simulink model "grid_afe_n"  (R2026a)
settings: Solver=ode23tb  StopTime=simlength  FixedStep=tc  MaxStep=glb_time.tc
values from neighbouring files (symbols this model uses):
  afe_ctrl = ctrl_afe_setup(glb_time.ts_afe, grid_emu.omega_grid_nom)    [init_model.m]
  afe_pwm_phase_shift_mod1 = 0    [init_model.m]
  afe_pwm_phase_shift_mod2 = 0    [init_model.m]
  afe_pwm_phase_shift_mod3 = 0    [init_model.m]
  afe_pwm_phase_shift_mod4 = 0    [init_model.m]
  filters = setup_global_filters(glb_time.ts_afe, glb_time.ts_inv, glb_time.ts_dab, glb_time.tc)    [init_model.m]
  frt_data = frt_settings(test_index, test_subindex, asymmetric_error_type,      enable_frt_1, enable_frt_2, start_time_LVRT, deepPOSxi, deepPOSeta, deepNEGxi, deepNEGeta)    [init_model.m]
  glb_time = timing_setup(fpwm_afe, trgo_afe, fpwm_inv, trgo_inv, fpwm_single_phase_inv, trgo_single_phase_inv, fpwm_dab, trgo_dab,      fpwm_psfbc, trgo_psfbc, fpwm_isop_rail, trgo_isop_rail, fpwm_cllc, trgo_cllc, t_measure, tc_factor, tc_decimation, delay_pwm, dead_time_afe,      dead_time_inv, dead_time_single_phase_inv, dead_time_dab, dead_time_psfbc, dead_time_isop_rail, dead_time_cllc)    [init_model.m]
  grid_emu = grid_three_phase_emulator('Dyn11', delta_star, grid_nominal_power, application_voltage, us1, us2, fgrid,                  eq_grid_inductance, eq_grid_resistance, eta, ucc, i1m, p_iron, n1, n2, core_area, core_length, mur,                  up_xi_pu_ref, up_eta_pu_ref, un_xi_pu_ref, un_eta_pu_ref)    [init_model.m]
  i_react_pos_ref_2 = -ixi_ref_mod1*tan(acos(0.95))    [init_model.m]
  i_react_pos_ref_3 = ixi_ref_mod1*tan(acos(0.95))    [init_model.m]
  ixi_ref_mod1 = -0.85    [init_model.m]
  ixi_ref_mod2 = -0.85    [init_model.m]
  ixi_ref_mod3 = -0.85    [init_model.m]
  ixi_ref_mod4 = -0.85    [init_model.m]
  ki_align = 18    [init_model.m]
  kp_align = 0.25    [init_model.m]
  lim_down_align = -0.05    [init_model.m]
  lim_up_align = 0.05    [init_model.m]
  mavarage_filter_frequency_base_order = 2    [init_model.m]
  time_gain_afe_module_1 = 1.0002    [init_model.m]
  time_gain_afe_module_2 = 1.0015    [init_model.m]
  time_gain_afe_module_3 = 0.9988    [init_model.m]
  time_gain_afe_module_4 = 1.0020    (= 1.002)    [init_model.m]
  time_i_react_pos_ref_1 = start_time_LVRT + error_length + 0.335    [init_model.m]
  time_i_react_pos_ref_2 = time_i_react_pos_ref_1 + 0.5    (= 0.5)    [init_model.m]
  u_cm_comp_mod1 = 0    [init_model.m]
  u_cm_comp_mod2 = -1    [init_model.m]
  u_cm_comp_mod3 = -1    [init_model.m]
  u_cm_comp_mod4 = -1    [init_model.m]
undefined symbols (not defined in the file or in its folder): hwdata, magnitude
libraries: fl_lib x113, nesl_utility x75, moving_average_filter x40, moving_average_filter_cc x32, sl_discontinuities x12, linear_double_integrator_observer_ccaller x8, discrete_time_low_pass_filter x4, threephase_inductor_lib x4, dclink_for_two_levels x4, three_phase_pwm_modulator x4, three_phase_inverter_ideal_switch_based_model x4, three_phase_inverter_igbt_advanced_thermal_model x4
(part 18 of 19)

== matlab function grid_afe_n/afe_abc_mod4/AFE_control/afe_control/FRT-VDE4110/FRT-Detection/LVRT_detector ==
  data: vxi_p input; vxi_n input; veta_n input; vxi_p_dot input; vxi_n_dot input; enable input; red_dyn_enabled input; pwr_lim_enable output; frt_exceeded output; reset input; frt_active output; frt_state output; red_dyn_active output
function [pwr_lim_enable, frt_exceeded, frt_active, frt_state, red_dyn_active]  = lvrt_detector(vxi_p,vxi_n,veta_n,vxi_p_dot,vxi_n_dot, enable, red_dyn_enabled, reset)

    persistent state count count2 state_pwr_lim
    
    LVRT_IDLE = 0;
    LVRT_ACTIVE = 1;
    LVRT_EXCEEDED = 2;
    
    PWR_LIM_DISABLED = 0;
    PWR_LIM_ENABLED  = 1;
    
    LVRT_VPOS_TH_LOW			= 0.85;
    LVRT_VPOS_TH_HIGH			= 1.15;
    LVRT_SEQ_DETECTION_HYST		= 0.1;
    LVRT_VNEG_TH				= 0.1;
    LVRT_VPOS_DOT_TH			= 2.0;
    LVRT_VNEG_DOT_TH			= 2.0;
    LVRT_VPOS_PWRLIM_TH			= 0.8;
    LVRT_VNEG_PWRLIM_TH			= 0.1;
    LVRT_PWRLIM_HYST			= 0.1;
    LVRT_VPOS_RED_DYN_TH        = 0.7;
    LVRT_VNEG_RED_DYN_TH        = 0.2;
    LVRT_TIME_HOLD_MAX          = 61000;
    
    RED_DYN_NOT_ACTIVE = 0;
    RED_DYN_ACTIVE     = 1;
        
    if isempty(state)
        state = LVRT_IDLE;
        state_pwr_lim = PWR_LIM_DISABLED;
        count = 0;
        count2 = 0;
    end

    vn = sqrt(vxi_n^2+veta_n^2);

    if enable == 1
        
        switch state
            
            case LVRT_IDLE
                if ((vxi_p > LVRT_VPOS_TH_HIGH || vxi_p < LVRT_VPOS_TH_LOW || vn > LVRT_VNEG_TH) ...
                     && (vxi_p_dot > LVRT_VPOS_DOT_TH || vxi_n_dot > LVRT_VNEG_DOT_TH) && ...
                     count2 > 1000)
                    state = LVRT_ACTIVE;
                end
                frt_active = 0;
                frt_exceeded = 0;
                count = 0;
                frt_state = LVRT_IDLE;
                state_pwr_lim = PWR_LIM_DISABLED;                  
                red_dyn_active = RED_DYN_NOT_ACTIVE;
                count2 = count2 + 1;

            case LVRT_ACTIVE
                count2 = 0;
                % LVRT condition not active anymore
                if (vxi_p >= LVRT_VPOS_TH_LOW  + LVRT_SEQ_DETECTION_HYST && ...
                    vxi_p <  LVRT_VPOS_TH_HIGH - LVRT_SEQ_DETECTION_HYST)
                    state = LVRT_IDLE;
                % LVRT exceeded
                elseif (count >= LVRT_TIME_HOLD_MAX)
                    state = LVRT_EXCEEDED;
                end
                
                % handle power limitation
                if (vxi_p < LVRT_VPOS_PWRLIM_TH || vn > LVRT_VNEG_PWRLIM_TH) 
                    state_pwr_lim = PWR_LIM_ENABLED;
                elseif (vxi_p > LVRT_VPOS_PWRLIM_TH + LVRT_PWRLIM_HYST && vn < LVRT_VPOS_PWRLIM_TH - LVRT_PWRLIM_HYST)
                    state_pwr_lim = PWR_LIM_DISABLED;                  
                end
                
                % handle reduced dynamic grid support
                if red_dyn_enabled && (vxi_p < LVRT_VPOS_RED_DYN_TH || vn > LVRT_VNEG_RED_DYN_TH)
                    red_dyn_active = RED_DYN_ACTIVE;
                else
                    red_dyn_active = RED_DYN_NOT_ACTIVE;
                end
                 
                frt_active = 1;
                frt_exceeded = 0;
                frt_state = LVRT_ACTIVE;
                
                count = count + 1;
            
            case LVRT_EXCEEDED

                if ((reset == 1) || (enable == 0))
                    state = LVRT_IDLE;
                else
                    state = LVRT_EXCEEDED;
                end
                
                frt_exceeded = 1;
                frt_active = 0; 
                frt_state = LVRT_EXCEEDED;
                red_dyn_active = RED_DYN_NOT_ACTIVE;
            
            otherwise
                state = LVRT_IDLE;
                frt_active = 0;
                frt_exceeded = 0;
                frt_state = LVRT_IDLE;
                red_dyn_active = RED_DYN_NOT_ACTIVE;
        end
        
        if state_pwr_lim == PWR_LIM_ENABLED
            pwr_lim_enable = 1;
        else
            pwr_lim_enable = 0;
        end      
    else
        state = LVRT_IDLE;
        frt_active = 0;
        pwr_lim_enable = 0;
        frt_exceeded = 0;
        frt_state = LVRT_IDLE;
        red_dyn_active = RED_DYN_NOT_ACTIVE;
    end
end

== matlab function grid_afe_n/afe_abc_mod1/AFE_control/afe_control/current_ctrl/current_transformation/alphabeta2xieta ==
  data: alpha input; xi output; beta input; gamma input; eta output
function [xi,eta] = alphabeta2xieta(alpha,beta,gamma)

    xi  =  alpha*cos(gamma) + beta*sin(gamma);
    eta = -alpha*sin(gamma) + beta*cos(gamma);

end

== matlab function grid_afe_n/afe_abc_mod4/AFE_control/afe_control/FRT-VDE4110/FRT-PosNegReactiveCurrentReferences/avg_flt_500ms/avg_flt_1 ==
  data: x input; y1 output; w input; ts input; enable input
function y1  = avg_flt(x,w,ts, enable)

    persistent x_int x_int_1 y_N N

    N = (1/(w/(2*pi)))/ts+1;

    if isempty(x_int)
        x_int_1 = 0;
        y_N = zeros(1,N);
        y1 = 0;
    end


    if enable == 1
        x_int = x * ts * w + x_int_1;
        x_int_1 = x_int;
        y_N(1,1) = x_int;
        y1 = 1/(2*pi)*((y_N(1,1) - y_N(1,N)));
        for i = 1:(N-1)
            y_N(1,N+1-i) = y_N(1,N-i); 
        end
    else
        y1 = 1/(2*pi)*((y_N(1,1) - y_N(1,N)));
    end
end

== matlab function grid_afe_n/afe_abc_mod4/AFE_control/afe_control/FRT-VDE4110/FRT-PosNegReactiveCurrentReferences/avg_flt_500ms1/avg_flt_1 ==
  data: x input; y1 output; w input; ts input; enable input
function y1  = avg_flt(x,w,ts, enable)

    persistent x_int x_int_1 y_N N

    N = (1/(w/(2*pi)))/ts+1;

    if isempty(x_int)
        x_int_1 = 0;
        y_N = zeros(1,N);
        y1 = 0;
    end


    if enable == 1
        x_int = x * ts * w + x_int_1;
        x_int_1 = x_int;
        y_N(1,1) = x_int;
        y1 = 1/(2*pi)*((y_N(1,1) - y_N(1,N)));
        for i = 1:(N-1)
            y_N(1,N+1-i) = y_N(1,N-i); 
        end
    else
        y1 = 1/(2*pi)*((y_N(1,1) - y_N(1,N)));
    end
end

== matlab function grid_afe_n/afe_abc_mod4/AFE_control/afe_control/FRT-VDE4110/FRT-PosNegReactiveCurrentReferences/avg_flt_500ms2/avg_flt_1 ==
  data: x input; y1 output; w input; ts input; enable input
function y1  = avg_flt(x,w,ts, enable)

    persistent x_int x_int_1 y_N N

    N = (1/(w/(2*pi)))/ts+1;

    if isempty(x_int)
        x_int_1 = 0;
        y_N = zeros(1,N);
        y1 = 0;
    end


    if enable == 1
        x_int = x * ts * w + x_int_1;
        x_int_1 = x_int;
        y_N(1,1) = x_int;
        y1 = 1/(2*pi)*((y_N(1,1) - y_N(1,N)));
        for i = 1:(N-1)
            y_N(1,N+1-i) = y_N(1,N-i); 
        end
    else
        y1 = 1/(2*pi)*((y_N(1,1) - y_N(1,N)));
    end
end

== matlab function grid_afe_n/afe_abc_mod4/AFE_control/afe_control/FRT-VDE4110/FRT-PosNegReactiveCurrentReferences/avg_flt_500ms3/avg_flt_1 ==
  data: x input; y1 output; w input; ts input; enable input
function y1  = avg_flt(x,w,ts, enable)

    persistent x_int x_int_1 y_N N

    N = (1/(w/(2*pi)))/ts+1;

    if isempty(x_int)
        x_int_1 = 0;
        y_N = zeros(1,N);
        y1 = 0;
    end


    if enable == 1
        x_int = x * ts * w + x_int_1;
        x_int_1 = x_int;
        y_N(1,1) = x_int;
        y1 = 1/(2*pi)*((y_N(1,1) - y_N(1,N)));
        for i = 1:(N-1)
            y_N(1,N+1-i) = y_N(1,N-i); 
        end
    else
        y1 = 1/(2*pi)*((y_N(1,1) - y_N(1,N)));
    end
end

== matlab function grid_afe_n/afe_abc_mod4/AFE_control/afe_control/current_ctrl/current_transformation/alphabeta2xieta ==
  data: alpha input; xi output; beta input; gamma input; eta output
function [xi,eta] = alphabeta2xieta(alpha,beta,gamma)

    xi  =  alpha*cos(gamma) + beta*sin(gamma);
    eta = -alpha*sin(gamma) + beta*cos(gamma);

end

== matlab function grid_afe_n/afe_abc_mod4/AFE_control/afe_control/current_ctrl/current_transformation/uvw2alphabeta ==
  data: u input; alpha output; v input; w input; beta output
function [alpha,beta] = uvw2alphabeta(u,v,w)

alpha = 2/3*(u - 1/2*v - 1/2*w);
beta  = 2/3*(sqrt(3)/2*(v - w));

end

== matlab function grid_afe_n/afe_abc_mod4/AFE_control/afe_control/current_ctrl/inner_current_ctrl/zero_current_ctrl/antiwind_up/MATLAB Function1 ==
  data: da input; das output; db input; dc input; scaling input; dbs output; dcs output
function [das, dbs, dcs] = fcn(da,db,dc,scaling)

das = da/scaling;
dbs = db/scaling;
dcs = dc/scaling;

== matlab function grid_afe_n/afe_abc_mod4/AFE_control/afe_control/current_ctrl/inner_current_ctrl/zero_current_ctrl/antiwind_up/MATLAB Function2 ==
  data: a input; alpha output; b input; c input; beta output; gamma output
function [alpha,beta, gamma] = abc2alphabeta(a,b,c)

alpha = 2/3*(a - 1/2*b - 1/2*c);
beta  = 1/sqrt(3)*(b - c);
gamma = (a+b+c)/3;

end

== matlab function grid_afe_n/afe_abc_mod4/AFE_control/afe_control/current_ctrl/xieta2abc/MATLAB Function2 ==
  data: alpha input; a output; beta input; b output; c output
function [a,b,c] = alphabeta2abc(alpha,beta)

a = alpha;
b = -(1/2)*alpha + sqrt(3)/2*beta;
c = -(1/2)*alpha - sqrt(3)/2*beta;

end

== matlab function grid_afe_n/afe_abc_mod4/AFE_control/afe_control/current_ctrl/xieta2abc/Negative Sequence ==
  data: xi input; alpha output; eta input; phase input; beta output
function [alpha,beta] = neg2alphabeta(xi,eta,phase)

    alpha = xi*cos(phase)  + eta*sin(phase);
    beta  = -xi*sin(phase) + eta*cos(phase);

end

== matlab function grid_afe_n/afe_abc_mod1/AFE_control/afe_control/grid_voltage_phase_lock_loops/FHT-PLL/pll_stageB/double_integrator_observer/bounder1 ==
  data: u input; y output
function y = bounder(u)
    
    y = -pi + mod(u+3*pi,2*pi);
    
end

== matlab function grid_afe_n/afe_abc_mod4/AFE_control/afe_control/current_ctrl/xieta2abc/Positive Sequence ==
  data: xi input; alpha output; eta input; phase input; beta output
function [alpha,beta] = pos2alphabeta(xi,eta,phase)

    alpha = xi*cos(phase) - eta*sin(phase);
    beta  = xi*sin(phase) + eta*cos(phase);

end

== matlab function grid_afe_n/afe_abc_mod4/AFE_control/afe_control/grid_current_sequences_and_reactive_pwr_ctrl/grid_current_sampling_and_alpha_beta_transformation/i_abc2alphabeta ==
  data: i_abc input; alpha output; beta output
function [alpha,beta] = abc2alphabeta(i_abc)

alpha = 2/3*(i_abc(1) - 1/2*i_abc(2) - 1/2*i_abc(3));
beta  = 1/sqrt(3)*(i_abc(2) - i_abc(3));

end

== matlab function grid_afe_n/afe_abc_mod4/AFE_control/afe_control/grid_current_sequences_and_reactive_pwr_ctrl/i_alphabeta2xieta/MATLAB Function ==
  data: alpha input; xi output; beta input; gamma input; eta output
function [xi,eta] = alphabeta2pos(alpha,beta,gamma)

    xi  =  alpha*cos(gamma) + beta*sin(gamma);
    eta = -alpha*sin(gamma) + beta*cos(gamma);

end

== matlab function grid_afe_n/afe_abc_mod4/AFE_control/afe_control/grid_current_sequences_and_reactive_pwr_ctrl/i_alphabeta2xieta/MATLAB Function1 ==
  data: alpha input; xi output; beta input; gamma input; eta output
function [xi,eta] = alphabeta2neg(alpha,beta,gamma)

    xi  = alpha*cos(gamma) - beta*sin(gamma);
    eta = alpha*sin(gamma) + beta*cos(gamma);

end

== matlab function grid_afe_n/afe_abc_mod4/AFE_control/afe_control/grid_voltage_phase_lock_loops/FHT-PLL/pll_stageA/filter_and_transformation/abc2alphabeta ==
  data: a input; alpha output; b input; c input; beta output
function [alpha,beta] = abc2alphabeta(a,b,c)

alpha = 2/3*(a - 1/2*b - 1/2*c);
beta  = 1/sqrt(3)*(b - c);

end

== matlab function grid_afe_n/afe_abc_mod4/AFE_control/afe_control/grid_voltage_phase_lock_loops/FHT-PLL/pll_stageA/sequences/alphabeta2xieta ==
  data: alpha input; xi output; beta input; gamma input; eta output
function [xi,eta] = alphabeta2xieta_pos(alpha,beta,gamma)

    xi  =  (alpha*cos(gamma) + beta*sin(gamma));
    eta = (-alpha*sin(gamma) + beta*cos(gamma));

end

== matlab function grid_afe_n/afe_abc_mod4/AFE_control/afe_control/grid_voltage_phase_lock_loops/FHT-PLL/pll_stageB/bounder1 ==
  data: u input; y output
function y = bounder(u)
    y = -pi + mod(u+3*pi,2*pi);
end

== matlab function grid_afe_n/afe_abc_mod2/AFE_control/afe_control/FRT-VDE4110/FRT-PosNegReactiveCurrentReferences/avg_flt_500ms/avg_flt_1 ==
  data: x input; y1 output; w input; ts input; enable input
function y1  = avg_flt(x,w,ts, enable)

    persistent x_int x_int_1 y_N N

    N = (1/(w/(2*pi)))/ts+1;

    if isempty(x_int)
        x_int_1 = 0;
        y_N = zeros(1,N);
        y1 = 0;
    end


    if enable == 1
        x_int = x * ts * w + x_int_1;
        x_int_1 = x_int;
        y_N(1,1) = x_int;
        y1 = 1/(2*pi)*((y_N(1,1) - y_N(1,N)));
        for i = 1:(N-1)
            y_N(1,N+1-i) = y_N(1,N-i); 
        end
    else
        y1 = 1/(2*pi)*((y_N(1,1) - y_N(1,N)));
    end
end

== matlab function grid_afe_n/afe_abc_mod4/AFE_control/afe_control/grid_voltage_phase_lock_loops/FHT-PLL/pll_stageB/double_integrator_observer/bounder1 ==
  data: u input; y output
function y = bounder(u)
    
    y = -pi + mod(u+3*pi,2*pi);
    
end

== matlab function grid_afe_n/afe_abc_mod4/AFE_control/afe_control/grid_voltage_phase_lock_loops/FHT-PLL/pll_stageB/double_integrator_observer/bounder2 ==
  data: u input; y output
function y = bounder(u)
    
    y = -pi + mod(u+3*pi,2*pi);
    
end

== matlab function grid_afe_n/afe_abc_mod4/AFE_control/afe_control/grid_voltage_phase_lock_loops/dq_pll/pll_stageA/mormalization_and_transformation/abc2alphabeta ==
  data: a input; alpha output; b input; c input; beta output
function [alpha,beta] = abc2alphabeta(a,b,c)

alpha = 2/3*(a - 1/2*b - 1/2*c);
beta  = 1/sqrt(3)*(b - c);

end

== matlab function grid_afe_n/afe_abc_mod4/AFE_control/afe_control/grid_voltage_phase_lock_loops/dq_pll/pll_stageA/sequences/alphabeta2xieta/alphabeta2xieta_neg ==
  data: alpha input; xi output; beta input; gamma input; eta output
function [xi,eta] = alphabeta2xieta_neg(alpha,beta,gamma)

    xi  = alpha*cos(gamma) - beta*sin(gamma);
    eta = alpha*sin(gamma) + beta*cos(gamma);

end

== matlab function grid_afe_n/afe_abc_mod4/AFE_control/afe_control/grid_voltage_phase_lock_loops/dq_pll/pll_stageA/sequences/alphabeta2xieta/alphabeta2xieta_pos ==
  data: alpha input; xi output; beta input; gamma input; eta output
function [xi,eta] = alphabeta2xieta_pos(alpha,beta,gamma)

    xi  =  alpha*cos(gamma) + beta*sin(gamma);
    eta = -alpha*sin(gamma) + beta*cos(gamma);

end

== matlab function grid_afe_n/afe_abc_mod4/AFE_control/afe_control/grid_voltage_phase_lock_loops/dq_pll/pll_stageB/bounder1 ==
  data: u input; y output
function y = bounder(u)
    y = -pi + mod(u+3*pi,2*pi);
end

== matlab function grid_afe_n/afe_abc_mod4/AFE_control/afe_control/grid_voltage_phase_lock_loops/dq_pll/pll_stageB/double_integrator_observer/bounder1 ==
  data: u input; y output
function y = bounder(u)
    
    y = -pi + mod(u+3*pi,2*pi);
    
end

== matlab function grid_afe_n/afe_abc_mod4/AFE_control/afe_control/grid_voltage_phase_lock_loops/dq_pll/pll_stageB/double_integrator_observer/bounder2 ==
  data: u input; y output
function y = bounder(u)
    
    y = -pi + mod(u+3*pi,2*pi);
    
end

== matlab function grid_afe_n/afe_abc_mod4/AFE_control/afe_control/grid_voltage_sequences/grid_voltage_sampling_and_alpha_beta_transformation/v_abc2alphabeta ==
  data: v_abc input; alpha output; beta output
function [alpha,beta] = abc2alphabeta(v_abc)

alpha = 2/3*(v_abc(1) - 1/2*v_abc(2) - 1/2*v_abc(3));
beta  = 1/sqrt(3)*(v_abc(2) - v_abc(3));

end

== matlab function grid_afe_n/afe_abc_mod4/AFE_control/afe_control/grid_voltage_sequences/v_alphabeta2xieta/MATLAB Function ==
  data: alpha input; xi output; beta input; gamma input; eta output
function [xi,eta] = alphabeta2pos(alpha,beta,gamma)

    xi  =  alpha*cos(gamma) + beta*sin(gamma);
    eta = -alpha*sin(gamma) + beta*cos(gamma);

end

== matlab function grid_afe_n/afe_abc_mod4/AFE_control/afe_control/grid_voltage_sequences/v_alphabeta2xieta/MATLAB Function1 ==
  data: alpha input; xi output; beta input; gamma input; eta output
function [xi,eta] = alphabeta2neg(alpha,beta,gamma)

    xi  = alpha*cos(gamma) - beta*sin(gamma);
    eta = alpha*sin(gamma) + beta*cos(gamma);

end

== matlab function grid_afe_n/afe_abc_mod4/AFE_control/afe_control/islanding_mode_detector/MATLAB Function ==
  data: alpha input; xi output; beta input; gamma input; eta output
function [xi,eta] = alphabeta2pos(alpha,beta,gamma)

    xi  =  alpha*cos(gamma) + beta*sin(gamma);
    eta = -alpha*sin(gamma) + beta*cos(gamma);

end

== matlab function grid_afe_n/afe_abc_mod2/AFE_control/afe_control/FRT-VDE4110/FRT-PosNegReactiveCurrentReferences/avg_flt_500ms1/avg_flt_1 ==
  data: x input; y1 output; w input; ts input; enable input
function y1  = avg_flt(x,w,ts, enable)

    persistent x_int x_int_1 y_N N

    N = (1/(w/(2*pi)))/ts+1;

    if isempty(x_int)
        x_int_1 = 0;
        y_N = zeros(1,N);
        y1 = 0;
    end


    if enable == 1
        x_int = x * ts * w + x_int_1;
        x_int_1 = x_int;
        y_N(1,1) = x_int;
        y1 = 1/(2*pi)*((y_N(1,1) - y_N(1,N)));
        for i = 1:(N-1)
            y_N(1,N+1-i) = y_N(1,N-i); 
        end
    else
        y1 = 1/(2*pi)*((y_N(1,1) - y_N(1,N)));
    end
end

== matlab function grid_afe_n/afe_abc_mod4/AFE_control/afe_control/islanding_mode_detector/bounder ==
  data: u input; y output
function y = bounder(u)
    
    u = -pi + mod(u+3*pi,2*pi);
    
    y = u;
end

== matlab function grid_afe_n/afe_abc_mod1/AFE_control/afe_control/FRT-VDE4110/FRT-Detection/LVRT_detector ==
  data: vxi_p input; vxi_n input; veta_n input; vxi_p_dot input; vxi_n_dot input; enable input; red_dyn_enabled input; pwr_lim_enable output; frt_exceeded output; reset input; frt_active output; frt_state output; red_dyn_active output
function [pwr_lim_enable, frt_exceeded, frt_active, frt_state, red_dyn_active]  = lvrt_detector(vxi_p,vxi_n,veta_n,vxi_p_dot,vxi_n_dot, enable, red_dyn_enabled, reset)

    persistent state count count2 state_pwr_lim
    
    LVRT_IDLE = 0;
    LVRT_ACTIVE = 1;
    LVRT_EXCEEDED = 2;
    
    PWR_LIM_DISABLED = 0;
    PWR_LIM_ENABLED  = 1;
    
    LVRT_VPOS_TH_LOW			= 0.85;
    LVRT_VPOS_TH_HIGH			= 1.15;
    LVRT_SEQ_DETECTION_HYST		= 0.1;
    LVRT_VNEG_TH				= 0.1;
    LVRT_VPOS_DOT_TH			= 2.0;
    LVRT_VNEG_DOT_TH			= 2.0;
    LVRT_VPOS_PWRLIM_TH			= 0.8;
    LVRT_VNEG_PWRLIM_TH			= 0.1;
    LVRT_PWRLIM_HYST			= 0.1;
    LVRT_VPOS_RED_DYN_TH        = 0.7;
    LVRT_VNEG_RED_DYN_TH        = 0.2;
    LVRT_TIME_HOLD_MAX          = 61000;
    
    RED_DYN_NOT_ACTIVE = 0;
    RED_DYN_ACTIVE     = 1;
        
    if isempty(state)
        state = LVRT_IDLE;
        state_pwr_lim = PWR_LIM_DISABLED;
        count = 0;
        count2 = 0;
    end

    vn = sqrt(vxi_n^2+veta_n^2);

    if enable == 1
        
        switch state
            
            case LVRT_IDLE
                if ((vxi_p > LVRT_VPOS_TH_HIGH || vxi_p < LVRT_VPOS_TH_LOW || vn > LVRT_VNEG_TH) ...
                     && (vxi_p_dot > LVRT_VPOS_DOT_TH || vxi_n_dot > LVRT_VNEG_DOT_TH) && ...
                     count2 > 1000)
                    state = LVRT_ACTIVE;
                end
                frt_active = 0;
                frt_exceeded = 0;
                count = 0;
                frt_state = LVRT_IDLE;
                state_pwr_lim = PWR_LIM_DISABLED;                  
                red_dyn_active = RED_DYN_NOT_ACTIVE;
                count2 = count2 + 1;

            case LVRT_ACTIVE
                count2 = 0;
                % LVRT condition not active anymore
                if (vxi_p >= LVRT_VPOS_TH_LOW  + LVRT_SEQ_DETECTION_HYST && ...
                    vxi_p <  LVRT_VPOS_TH_HIGH - LVRT_SEQ_DETECTION_HYST)
                    state = LVRT_IDLE;
                % LVRT exceeded
                elseif (count >= LVRT_TIME_HOLD_MAX)
                    state = LVRT_EXCEEDED;
                end
                
                % handle power limitation
                if (vxi_p < LVRT_VPOS_PWRLIM_TH || vn > LVRT_VNEG_PWRLIM_TH) 
                    state_pwr_lim = PWR_LIM_ENABLED;
                elseif (vxi_p > LVRT_VPOS_PWRLIM_TH + LVRT_PWRLIM_HYST && vn < LVRT_VPOS_PWRLIM_TH - LVRT_PWRLIM_HYST)
                    state_pwr_lim = PWR_LIM_DISABLED;                  
                end
                
                % handle reduced dynamic grid support
                if red_dyn_enabled && (vxi_p < LVRT_VPOS_RED_DYN_TH || vn > LVRT_VNEG_RED_DYN_TH)
                    red_dyn_active = RED_DYN_ACTIVE;
                else
                    red_dyn_active = RED_DYN_NOT_ACTIVE;
                end
                 
                frt_active = 1;
                frt_exceeded = 0;
                frt_state = LVRT_ACTIVE;
                
                count = count + 1;
            
            case LVRT_EXCEEDED

                if ((reset == 1) || (enable == 0))
                    state = LVRT_IDLE;
                else
                    state = LVRT_EXCEEDED;
                end
                
                frt_exceeded = 1;
                frt_active = 0; 
                frt_state = LVRT_EXCEEDED;
                red_dyn_active = RED_DYN_NOT_ACTIVE;
            
            otherwise
                state = LVRT_IDLE;
                frt_active = 0;
                frt_exceeded = 0;
                frt_state = LVRT_IDLE;
                red_dyn_active = RED_DYN_NOT_ACTIVE;
        end
        
        if state_pwr_lim == PWR_LIM_ENABLED
            pwr_lim_enable = 1;
        else
            pwr_lim_enable = 0;
        end      
    else
        state = LVRT_IDLE;
        frt_active = 0;
        pwr_lim_enable = 0;
        frt_exceeded = 0;
        frt_state = LVRT_IDLE;
        red_dyn_active = RED_DYN_NOT_ACTIVE;
    end
end

== matlab function grid_afe_n/afe_abc_mod2/AFE_control/afe_control/FRT-VDE4110/FRT-PosNegReactiveCurrentReferences/avg_flt_500ms2/avg_flt_1 ==
  data: x input; y1 output; w input; ts input; enable input
function y1  = avg_flt(x,w,ts, enable)

    persistent x_int x_int_1 y_N N

    N = (1/(w/(2*pi)))/ts+1;

    if isempty(x_int)
        x_int_1 = 0;
        y_N = zeros(1,N);
        y1 = 0;
    end


    if enable == 1
        x_int = x * ts * w + x_int_1;
        x_int_1 = x_int;
        y_N(1,1) = x_int;
        y1 = 1/(2*pi)*((y_N(1,1) - y_N(1,N)));
        for i = 1:(N-1)
            y_N(1,N+1-i) = y_N(1,N-i); 
        end
    else
        y1 = 1/(2*pi)*((y_N(1,1) - y_N(1,N)));
    end
end

== matlab function grid_afe_n/afe_abc_mod1/AFE_control/afe_control/grid_voltage_phase_lock_loops/FHT-PLL/pll_stageB/double_integrator_observer/bounder2 ==
  data: u input; y output
function y = bounder(u)
    
    y = -pi + mod(u+3*pi,2*pi);
    
end

== matlab function grid_afe_n/afe_abc_mod1/AFE_control/afe_control/grid_voltage_phase_lock_loops/FHT-PLL_simulink/pll_stageA/filter_and_transformation/abc2alphabeta ==
  data: a input; alpha output; b input; c input; beta output
function [alpha,beta] = abc2alphabeta(a,b,c)

alpha = 2/3*(a - 1/2*b - 1/2*c);
beta  = 1/sqrt(3)*(b - c);

end

== matlab function grid_afe_n/afe_abc_mod2/AFE_control/afe_control/FRT-VDE4110/FRT-PosNegReactiveCurrentReferences/avg_flt_500ms3/avg_flt_1 ==
  data: x input; y1 output; w input; ts input; enable input
function y1  = avg_flt(x,w,ts, enable)

    persistent x_int x_int_1 y_N N

    N = (1/(w/(2*pi)))/ts+1;

    if isempty(x_int)
        x_int_1 = 0;
        y_N = zeros(1,N);
        y1 = 0;
    end


    if enable == 1
        x_int = x * ts * w + x_int_1;
        x_int_1 = x_int;
        y_N(1,1) = x_int;
        y1 = 1/(2*pi)*((y_N(1,1) - y_N(1,N)));
        for i = 1:(N-1)
            y_N(1,N+1-i) = y_N(1,N-i); 
        end
    else
        y1 = 1/(2*pi)*((y_N(1,1) - y_N(1,N)));
    end
end

== matlab function grid_afe_n/afe_abc_mod1/AFE_control/afe_control/grid_voltage_phase_lock_loops/FHT-PLL_simulink/pll_stageA/sequences/alphabeta2xieta ==
  data: alpha input; xi output; beta input; gamma input; eta output
function [xi,eta] = alphabeta2xieta_pos(alpha,beta,gamma)

    xi  =  (alpha*cos(gamma) + beta*sin(gamma));
    eta = (-alpha*sin(gamma) + beta*cos(gamma));

end

== matlab function grid_afe_n/afe_abc_mod1/AFE_control/afe_control/grid_voltage_phase_lock_loops/FHT-PLL_simulink/pll_stageB/bounder1 ==
  data: u input; y output
function y = bounder(u)
    y = -pi + mod(u+3*pi,2*pi);
end

== matlab function grid_afe_n/afe_abc_mod1/AFE_control/afe_control/grid_voltage_phase_lock_loops/FHT-PLL_simulink/pll_stageB/double_integrator_observer/bounder1 ==
  data: u input; y output
function y = bounder(u)
    
    y = -pi + mod(u+3*pi,2*pi);
    
end

== matlab function grid_afe_n/afe_abc_mod1/AFE_control/afe_control/grid_voltage_phase_lock_loops/dq_pll/pll_stageB/double_integrator_observer/bounder1 ==
  data: u input; y output
function y = bounder(u)
    
    y = -pi + mod(u+3*pi,2*pi);
    
end

== matlab function grid_afe_n/afe_abc_mod1/AFE_control/afe_control/grid_voltage_phase_lock_loops/dq_pll/pll_stageA/mormalization_and_transformation/abc2alphabeta ==
  data: a input; alpha output; b input; c input; beta output
function [alpha,beta] = abc2alphabeta(a,b,c)

alpha = 2/3*(a - 1/2*b - 1/2*c);
beta  = 1/sqrt(3)*(b - c);

end

== matlab function grid_afe_n/afe_abc_mod1/AFE_control/afe_control/grid_voltage_phase_lock_loops/dq_pll/pll_stageA/sequences/alphabeta2xieta/alphabeta2xieta_neg ==
  data: alpha input; xi output; beta input; gamma input; eta output
function [xi,eta] = alphabeta2xieta_neg(alpha,beta,gamma)

    xi  = alpha*cos(gamma) - beta*sin(gamma);
    eta = alpha*sin(gamma) + beta*cos(gamma);

end

== matlab function grid_afe_n/afe_abc_mod1/AFE_control/afe_control/grid_voltage_phase_lock_loops/dq_pll/pll_stageA/sequences/alphabeta2xieta/alphabeta2xieta_pos ==
  data: alpha input; xi output; beta input; gamma input; eta output
function [xi,eta] = alphabeta2xieta_pos(alpha,beta,gamma)

    xi  =  alpha*cos(gamma) + beta*sin(gamma);
    eta = -alpha*sin(gamma) + beta*cos(gamma);

end

== matlab function grid_afe_n/afe_abc_mod2/AFE_control/afe_control/current_ctrl/current_transformation/alphabeta2xieta ==
  data: alpha input; xi output; beta input; gamma input; eta output
function [xi,eta] = alphabeta2xieta(alpha,beta,gamma)

    xi  =  alpha*cos(gamma) + beta*sin(gamma);
    eta = -alpha*sin(gamma) + beta*cos(gamma);

end

== matlab function grid_afe_n/afe_abc_mod2/AFE_control/afe_control/current_ctrl/current_transformation/uvw2alphabeta ==
  data: u input; alpha output; v input; w input; beta output
function [alpha,beta] = uvw2alphabeta(u,v,w)

alpha = 2/3*(u - 1/2*v - 1/2*w);
beta  = 2/3*(sqrt(3)/2*(v - w));

end

== matlab function grid_afe_n/afe_abc_mod1/AFE_control/afe_control/FRT-VDE4110/FRT-PosNegReactiveCurrentReferences/avg_flt_500ms/avg_flt_1 ==
  data: x input; y1 output; w input; ts input; enable input
function y1  = avg_flt(x,w,ts, enable)

    persistent x_int x_int_1 y_N N

    N = (1/(w/(2*pi)))/ts+1;

    if isempty(x_int)
        x_int_1 = 0;
        y_N = zeros(1,N);
        y1 = 0;
    end


    if enable == 1
        x_int = x * ts * w + x_int_1;
        x_int_1 = x_int;
        y_N(1,1) = x_int;
        y1 = 1/(2*pi)*((y_N(1,1) - y_N(1,N)));
        for i = 1:(N-1)
            y_N(1,N+1-i) = y_N(1,N-i); 
        end
    else
        y1 = 1/(2*pi)*((y_N(1,1) - y_N(1,N)));
    end
end

== matlab function grid_afe_n/afe_abc_mod1/AFE_control/afe_control/islanding_mode_detector/MATLAB Function ==
  data: alpha input; xi output; beta input; gamma input; eta output
function [xi,eta] = alphabeta2pos(alpha,beta,gamma)

    xi  =  alpha*cos(gamma) + beta*sin(gamma);
    eta = -alpha*sin(gamma) + beta*cos(gamma);

end

== matlab function grid_afe_n/afe_abc_mod1/AFE_control/afe_control/islanding_mode_detector/bounder ==
  data: u input; y output
function y = bounder(u)
    
    u = -pi + mod(u+3*pi,2*pi);
    
    y = u;
end

== matlab function grid_afe_n/afe_abc_mod1/AFE_control/afe_control/grid_voltage_phase_lock_loops/dq_pll/pll_stageB/double_integrator_observer/bounder2 ==
  data: u input; y output
function y = bounder(u)
    
    y = -pi + mod(u+3*pi,2*pi);
    
end

== matlab function grid_afe_n/afe_abc_mod2/AFE_control/afe_control/current_ctrl/inner_current_ctrl/zero_current_ctrl/antiwind_up/MATLAB Function1 ==
  data: da input; das output; db input; dc input; scaling input; dbs output; dcs output
function [das, dbs, dcs] = fcn(da,db,dc,scaling)

das = da/scaling;
dbs = db/scaling;
dcs = dc/scaling;

== matlab function grid_afe_n/afe_abc_mod2/AFE_control/afe_control/current_ctrl/inner_current_ctrl/zero_current_ctrl/antiwind_up/MATLAB Function2 ==
  data: a input; alpha output; b input; c input; beta output; gamma output
function [alpha,beta, gamma] = abc2alphabeta(a,b,c)

alpha = 2/3*(a - 1/2*b - 1/2*c);
beta  = 1/sqrt(3)*(b - c);
gamma = (a+b+c)/3;

end

== matlab function grid_afe_n/afe_abc_mod1/AFE_control/afe_control/current_ctrl/inner_current_ctrl/zero_current_ctrl/antiwind_up/MATLAB Function1 ==
  data: da input; das output; db input; dc input; scaling input; dbs output; dcs output
function [das, dbs, dcs] = fcn(da,db,dc,scaling)

das = da/scaling;
dbs = db/scaling;
dcs = dc/scaling;

== matlab function grid_afe_n/afe_abc_mod2/AFE_control/afe_control/current_ctrl/xieta2abc/MATLAB Function2 ==
  data: alpha input; a output; beta input; b output; c output
function [a,b,c] = alphabeta2abc(alpha,beta)

a = alpha;
b = -(1/2)*alpha + sqrt(3)/2*beta;
c = -(1/2)*alpha - sqrt(3)/2*beta;

end

== matlab function grid_afe_n/afe_abc_mod1/AFE_control/afe_control/FRT-VDE4110/FRT-PosNegReactiveCurrentReferences/avg_flt_500ms1/avg_flt_1 ==
  data: x input; y1 output; w input; ts input; enable input
function y1  = avg_flt(x,w,ts, enable)

    persistent x_int x_int_1 y_N N

    N = (1/(w/(2*pi)))/ts+1;

    if isempty(x_int)
        x_int_1 = 0;
        y_N = zeros(1,N);
        y1 = 0;
    end


    if enable == 1
        x_int = x * ts * w + x_int_1;
        x_int_1 = x_int;
        y_N(1,1) = x_int;
        y1 = 1/(2*pi)*((y_N(1,1) - y_N(1,N)));
        for i = 1:(N-1)
            y_N(1,N+1-i) = y_N(1,N-i); 
        end
    else
        y1 = 1/(2*pi)*((y_N(1,1) - y_N(1,N)));
    end
end

== matlab function grid_afe_n/afe_abc_mod1/AFE_control/afe_control/FRT-VDE4110/FRT-PosNegReactiveCurrentReferences/avg_flt_500ms2/avg_flt_1 ==
  data: x input; y1 output; w input; ts input; enable input
function y1  = avg_flt(x,w,ts, enable)

    persistent x_int x_int_1 y_N N

    N = (1/(w/(2*pi)))/ts+1;

    if isempty(x_int)
        x_int_1 = 0;
        y_N = zeros(1,N);
        y1 = 0;
    end


    if enable == 1
        x_int = x * ts * w + x_int_1;
        x_int_1 = x_int;
        y_N(1,1) = x_int;
        y1 = 1/(2*pi)*((y_N(1,1) - y_N(1,N)));
        for i = 1:(N-1)
            y_N(1,N+1-i) = y_N(1,N-i); 
        end
    else
        y1 = 1/(2*pi)*((y_N(1,1) - y_N(1,N)));
    end
end

== matlab function grid_afe_n/afe_abc_mod1/AFE_control/afe_control/FRT-VDE4110/FRT-PosNegReactiveCurrentReferences/avg_flt_500ms3/avg_flt_1 ==
  data: x input; y1 output; w input; ts input; enable input
function y1  = avg_flt(x,w,ts, enable)

    persistent x_int x_int_1 y_N N

    N = (1/(w/(2*pi)))/ts+1;

    if isempty(x_int)
        x_int_1 = 0;
        y_N = zeros(1,N);
        y1 = 0;
    end


    if enable == 1
        x_int = x * ts * w + x_int_1;
        x_int_1 = x_int;
        y_N(1,1) = x_int;
        y1 = 1/(2*pi)*((y_N(1,1) - y_N(1,N)));
        for i = 1:(N-1)
            y_N(1,N+1-i) = y_N(1,N-i); 
        end
    else
        y1 = 1/(2*pi)*((y_N(1,1) - y_N(1,N)));
    end
end

== matlab function grid_afe_n/afe_abc_mod1/AFE_control/afe_control/grid_voltage_sequences/v_alphabeta2xieta/MATLAB Function ==
  data: alpha input; xi output; beta input; gamma input; eta output
function [xi,eta] = alphabeta2pos(alpha,beta,gamma)

    xi  =  alpha*cos(gamma) + beta*sin(gamma);
    eta = -alpha*sin(gamma) + beta*cos(gamma);

end

== matlab function grid_afe_n/afe_abc_mod1/AFE_control/afe_control/grid_voltage_sequences/v_alphabeta2xieta/MATLAB Function1 ==
  data: alpha input; xi output; beta input; gamma input; eta output
function [xi,eta] = alphabeta2neg(alpha,beta,gamma)

    xi  = alpha*cos(gamma) - beta*sin(gamma);
    eta = alpha*sin(gamma) + beta*cos(gamma);

end

== matlab function grid_afe_n/afe_abc_mod1/AFE_control/afe_control/grid_voltage_sequences/grid_voltage_sampling_and_alpha_beta_transformation/v_abc2alphabeta ==
  data: v_abc input; alpha output; beta output
function [alpha,beta] = abc2alphabeta(v_abc)

alpha = 2/3*(v_abc(1) - 1/2*v_abc(2) - 1/2*v_abc(3));
beta  = 1/sqrt(3)*(v_abc(2) - v_abc(3));

end

== matlab function grid_afe_n/afe_abc_mod1/AFE_control/afe_control/grid_current_sequences_and_reactive_pwr_ctrl/i_alphabeta2xieta/MATLAB Function ==
  data: alpha input; xi output; beta input; gamma input; eta output
function [xi,eta] = alphabeta2pos(alpha,beta,gamma)

    xi  =  alpha*cos(gamma) + beta*sin(gamma);
    eta = -alpha*sin(gamma) + beta*cos(gamma);

end

== matlab function grid_afe_n/afe_abc_mod1/AFE_control/afe_control/grid_current_sequences_and_reactive_pwr_ctrl/i_alphabeta2xieta/MATLAB Function1 ==
  data: alpha input; xi output; beta input; gamma input; eta output
function [xi,eta] = alphabeta2neg(alpha,beta,gamma)

    xi  = alpha*cos(gamma) - beta*sin(gamma);
    eta = alpha*sin(gamma) + beta*cos(gamma);

end

== matlab function grid_afe_n/afe_abc_mod1/AFE_control/afe_control/grid_current_sequences_and_reactive_pwr_ctrl/grid_current_sampling_and_alpha_beta_transformation/i_abc2alphabeta ==
  data: i_abc input; alpha output; beta output
function [alpha,beta] = abc2alphabeta(i_abc)

alpha = 2/3*(i_abc(1) - 1/2*i_abc(2) - 1/2*i_abc(3));
beta  = 1/sqrt(3)*(i_abc(2) - i_abc(3));

end

== matlab function grid_afe_n/afe_abc_mod2/AFE_control/afe_control/current_ctrl/xieta2abc/Negative Sequence ==
  data: xi input; alpha output; eta input; phase input; beta output
function [alpha,beta] = neg2alphabeta(xi,eta,phase)

    alpha = xi*cos(phase)  + eta*sin(phase);
    beta  = -xi*sin(phase) + eta*cos(phase);

end

== matlab function grid_afe_n/afe_abc_mod1/AFE_control/afe_control/current_ctrl/inner_current_ctrl/zero_current_ctrl/antiwind_up/MATLAB Function2 ==
  data: a input; alpha output; b input; c input; beta output; gamma output
function [alpha,beta, gamma] = abc2alphabeta(a,b,c)

alpha = 2/3*(a - 1/2*b - 1/2*c);
beta  = 1/sqrt(3)*(b - c);
gamma = (a+b+c)/3;

end

== matlab function grid_afe_n/afe_abc_mod1/AFE_control/afe_control/current_ctrl/xieta2abc/MATLAB Function2 ==
  data: alpha input; a output; beta input; b output; c output
function [a,b,c] = alphabeta2abc(alpha,beta)

a = alpha;
b = -(1/2)*alpha + sqrt(3)/2*beta;
c = -(1/2)*alpha - sqrt(3)/2*beta;

end

== matlab function grid_afe_n/afe_abc_mod1/AFE_control/afe_control/current_ctrl/xieta2abc/Negative Sequence ==
  data: xi input; alpha output; eta input; phase input; beta output
function [alpha,beta] = neg2alphabeta(xi,eta,phase)

    alpha = xi*cos(phase)  + eta*sin(phase);
    beta  = -xi*sin(phase) + eta*cos(phase);

end

== matlab function grid_afe_n/afe_abc_mod1/AFE_control/afe_control/current_ctrl/xieta2abc/Positive Sequence ==
  data: xi input; alpha output; eta input; phase input; beta output
function [alpha,beta] = pos2alphabeta(xi,eta,phase)

    alpha = xi*cos(phase) - eta*sin(phase);
    beta  = xi*sin(phase) + eta*cos(phase);

end

== matlab function grid_afe_n/afe_abc_mod1/AFE_control/afe_control/grid_voltage_phase_lock_loops/dq_pll/pll_stageB/bounder1 ==
  data: u input; y output
function y = bounder(u)
    y = -pi + mod(u+3*pi,2*pi);
end

== matlab function grid_afe_n/afe_abc_mod2/AFE_control/afe_control/current_ctrl/xieta2abc/Positive Sequence ==
  data: xi input; alpha output; eta input; phase input; beta output
function [alpha,beta] = pos2alphabeta(xi,eta,phase)

    alpha = xi*cos(phase) - eta*sin(phase);
    beta  = xi*sin(phase) + eta*cos(phase);

end

== matlab function grid_afe_n/afe_abc_mod2/AFE_control/afe_control/grid_current_sequences_and_reactive_pwr_ctrl/grid_current_sampling_and_alpha_beta_transformation/i_abc2alphabeta ==
  data: i_abc input; alpha output; beta output
function [alpha,beta] = abc2alphabeta(i_abc)

alpha = 2/3*(i_abc(1) - 1/2*i_abc(2) - 1/2*i_abc(3));
beta  = 1/sqrt(3)*(i_abc(2) - i_abc(3));

end

== matlab function grid_afe_n/afe_abc_mod1/AFE_control/afe_control/grid_voltage_phase_lock_loops/FHT-PLL_simulink/pll_stageB/double_integrator_observer/bounder2 ==
  data: u input; y output
function y = bounder(u)
    
    y = -pi + mod(u+3*pi,2*pi);
    
end

== matlab function grid_afe_n/afe_abc_mod2/AFE_control/afe_control/grid_voltage_phase_lock_loops/FHT-PLL_simulink/pll_stageA/filter_and_transformation/abc2alphabeta ==
  data: a input; alpha output; b input; c input; beta output
function [alpha,beta] = abc2alphabeta(a,b,c)

alpha = 2/3*(a - 1/2*b - 1/2*c);
beta  = 1/sqrt(3)*(b - c);

end

== matlab function grid_afe_n/afe_abc_mod2/AFE_control/afe_control/grid_voltage_phase_lock_loops/FHT-PLL_simulink/pll_stageA/sequences/alphabeta2xieta ==
  data: alpha input; xi output; beta input; gamma input; eta output
function [xi,eta] = alphabeta2xieta_pos(alpha,beta,gamma)

    xi  =  (alpha*cos(gamma) + beta*sin(gamma));
    eta = (-alpha*sin(gamma) + beta*cos(gamma));

end

== matlab function grid_afe_n/afe_abc_mod2/AFE_control/afe_control/grid_voltage_phase_lock_loops/FHT-PLL_simulink/pll_stageB/bounder1 ==
  data: u input; y output
function y = bounder(u)
    y = -pi + mod(u+3*pi,2*pi);
end

== matlab function grid_afe_n/afe_abc_mod2/AFE_control/afe_control/grid_voltage_phase_lock_loops/FHT-PLL_simulink/pll_stageB/double_integrator_observer/bounder1 ==
  data: u input; y output
function y = bounder(u)
    
    y = -pi + mod(u+3*pi,2*pi);
    
end

== matlab function grid_afe_n/afe_abc_mod2/AFE_control/afe_control/grid_current_sequences_and_reactive_pwr_ctrl/i_alphabeta2xieta/MATLAB Function ==
  data: alpha input; xi output; beta input; gamma input; eta output
function [xi,eta] = alphabeta2pos(alpha,beta,gamma)

    xi  =  alpha*cos(gamma) + beta*sin(gamma);
    eta = -alpha*sin(gamma) + beta*cos(gamma);

end

== matlab function grid_afe_n/afe_abc_mod1/AFE_control/afe_control/grid_voltage_phase_lock_loops/FHT-PLL/pll_stageA/filter_and_transformation/abc2alphabeta ==
  data: a input; alpha output; b input; c input; beta output
function [alpha,beta] = abc2alphabeta(a,b,c)

alpha = 2/3*(a - 1/2*b - 1/2*c);
beta  = 1/sqrt(3)*(b - c);

end

== matlab function grid_afe_n/afe_abc_mod2/AFE_control/afe_control/grid_current_sequences_and_reactive_pwr_ctrl/i_alphabeta2xieta/MATLAB Function1 ==
  data: alpha input; xi output; beta input; gamma input; eta output
function [xi,eta] = alphabeta2neg(alpha,beta,gamma)

    xi  = alpha*cos(gamma) - beta*sin(gamma);
    eta = alpha*sin(gamma) + beta*cos(gamma);

end

== matlab function grid_afe_n/afe_abc_mod2/AFE_control/afe_control/grid_voltage_phase_lock_loops/FHT-PLL_simulink/pll_stageB/double_integrator_observer/bounder2 ==
  data: u input; y output
function y = bounder(u)
    
    y = -pi + mod(u+3*pi,2*pi);
    
end

== matlab function grid_afe_n/afe_abc_mod3/AFE_control/afe_control/grid_voltage_phase_lock_loops/FHT-PLL_simulink/pll_stageA/filter_and_transformation/abc2alphabeta ==
  data: a input; alpha output; b input; c input; beta output
function [alpha,beta] = abc2alphabeta(a,b,c)

alpha = 2/3*(a - 1/2*b - 1/2*c);
beta  = 1/sqrt(3)*(b - c);

end

== matlab function grid_afe_n/afe_abc_mod3/AFE_control/afe_control/grid_voltage_phase_lock_loops/FHT-PLL_simulink/pll_stageA/sequences/alphabeta2xieta ==
  data: alpha input; xi output; beta input; gamma input; eta output
function [xi,eta] = alphabeta2xieta_pos(alpha,beta,gamma)

    xi  =  (alpha*cos(gamma) + beta*sin(gamma));
    eta = (-alpha*sin(gamma) + beta*cos(gamma));

end

== matlab function grid_afe_n/afe_abc_mod3/AFE_control/afe_control/grid_voltage_phase_lock_loops/FHT-PLL_simulink/pll_stageB/bounder1 ==
  data: u input; y output
function y = bounder(u)
    y = -pi + mod(u+3*pi,2*pi);
end

== matlab function grid_afe_n/afe_abc_mod3/AFE_control/afe_control/grid_voltage_phase_lock_loops/FHT-PLL_simulink/pll_stageB/double_integrator_observer/bounder1 ==
  data: u input; y output
function y = bounder(u)
    
    y = -pi + mod(u+3*pi,2*pi);
    
end

== matlab function grid_afe_n/afe_abc_mod3/AFE_control/afe_control/grid_voltage_phase_lock_loops/FHT-PLL_simulink/pll_stageB/double_integrator_observer/bounder2 ==
  data: u input; y output
function y = bounder(u)
    
    y = -pi + mod(u+3*pi,2*pi);
    
end

== matlab function grid_afe_n/afe_abc_mod4/AFE_control/afe_control/grid_voltage_phase_lock_loops/FHT-PLL_simulink/pll_stageA/filter_and_transformation/abc2alphabeta ==
  data: a input; alpha output; b input; c input; beta output
function [alpha,beta] = abc2alphabeta(a,b,c)

alpha = 2/3*(a - 1/2*b - 1/2*c);
beta  = 1/sqrt(3)*(b - c);

end

== matlab function grid_afe_n/afe_abc_mod4/AFE_control/afe_control/grid_voltage_phase_lock_loops/FHT-PLL_simulink/pll_stageA/sequences/alphabeta2xieta ==
  data: alpha input; xi output; beta input; gamma input; eta output
function [xi,eta] = alphabeta2xieta_pos(alpha,beta,gamma)

    xi  =  (alpha*cos(gamma) + beta*sin(gamma));
    eta = (-alpha*sin(gamma) + beta*cos(gamma));

end

== matlab function grid_afe_n/afe_abc_mod4/AFE_control/afe_control/grid_voltage_phase_lock_loops/FHT-PLL_simulink/pll_stageB/bounder1 ==
  data: u input; y output
function y = bounder(u)
    y = -pi + mod(u+3*pi,2*pi);
end

== matlab function grid_afe_n/afe_abc_mod2/AFE_control/afe_control/grid_voltage_phase_lock_loops/FHT-PLL/pll_stageA/filter_and_transformation/abc2alphabeta ==
  data: a input; alpha output; b input; c input; beta output
function [alpha,beta] = abc2alphabeta(a,b,c)

alpha = 2/3*(a - 1/2*b - 1/2*c);
beta  = 1/sqrt(3)*(b - c);

end

== matlab function grid_afe_n/afe_abc_mod1/AFE_control/afe_control/grid_voltage_phase_lock_loops/FHT-PLL/pll_stageA/sequences/alphabeta2xieta ==
  data: alpha input; xi output; beta input; gamma input; eta output
function [xi,eta] = alphabeta2xieta_pos(alpha,beta,gamma)

    xi  =  (alpha*cos(gamma) + beta*sin(gamma));
    eta = (-alpha*sin(gamma) + beta*cos(gamma));

end

== matlab function grid_afe_n/afe_abc_mod2/AFE_control/afe_control/grid_voltage_phase_lock_loops/FHT-PLL/pll_stageA/sequences/alphabeta2xieta ==
  data: alpha input; xi output; beta input; gamma input; eta output
function [xi,eta] = alphabeta2xieta_pos(alpha,beta,gamma)

    xi  =  (alpha*cos(gamma) + beta*sin(gamma));
    eta = (-alpha*sin(gamma) + beta*cos(gamma));

end

== matlab function grid_afe_n/afe_abc_mod2/AFE_control/afe_control/grid_voltage_phase_lock_loops/FHT-PLL/pll_stageB/bounder1 ==
  data: u input; y output
function y = bounder(u)
    y = -pi + mod(u+3*pi,2*pi);
end

== matlab function grid_afe_n/afe_abc_mod2/AFE_control/afe_control/grid_voltage_phase_lock_loops/FHT-PLL/pll_stageB/double_integrator_observer/bounder1 ==
  data: u input; y output
function y = bounder(u)
    
    y = -pi + mod(u+3*pi,2*pi);
    
end

== matlab function grid_afe_n/afe_abc_mod2/AFE_control/afe_control/grid_voltage_phase_lock_loops/FHT-PLL/pll_stageB/double_integrator_observer/bounder2 ==
  data: u input; y output
function y = bounder(u)
    
    y = -pi + mod(u+3*pi,2*pi);
    
end

== matlab function grid_afe_n/afe_abc_mod2/AFE_control/afe_control/grid_voltage_phase_lock_loops/dq_pll/pll_stageA/mormalization_and_transformation/abc2alphabeta ==
  data: a input; alpha output; b input; c input; beta output
function [alpha,beta] = abc2alphabeta(a,b,c)

alpha = 2/3*(a - 1/2*b - 1/2*c);
beta  = 1/sqrt(3)*(b - c);

end

== matlab function grid_afe_n/afe_abc_mod2/AFE_control/afe_control/grid_voltage_phase_lock_loops/dq_pll/pll_stageA/sequences/alphabeta2xieta/alphabeta2xieta_neg ==
  data: alpha input; xi output; beta input; gamma input; eta output
function [xi,eta] = alphabeta2xieta_neg(alpha,beta,gamma)

    xi  = alpha*cos(gamma) - beta*sin(gamma);
    eta = alpha*sin(gamma) + beta*cos(gamma);

end

== matlab function grid_afe_n/afe_abc_mod2/AFE_control/afe_control/grid_voltage_phase_lock_loops/dq_pll/pll_stageA/sequences/alphabeta2xieta/alphabeta2xieta_pos ==
  data: alpha input; xi output; beta input; gamma input; eta output
function [xi,eta] = alphabeta2xieta_pos(alpha,beta,gamma)

    xi  =  alpha*cos(gamma) + beta*sin(gamma);
    eta = -alpha*sin(gamma) + beta*cos(gamma);

end

== matlab function grid_afe_n/afe_abc_mod2/AFE_control/afe_control/grid_voltage_phase_lock_loops/dq_pll/pll_stageB/bounder1 ==
  data: u input; y output
function y = bounder(u)
    y = -pi + mod(u+3*pi,2*pi);
end

== matlab function grid_afe_n/afe_abc_mod2/AFE_control/afe_control/grid_voltage_phase_lock_loops/dq_pll/pll_stageB/double_integrator_observer/bounder1 ==
  data: u input; y output
function y = bounder(u)
    
    y = -pi + mod(u+3*pi,2*pi);
    
end

== matlab function grid_afe_n/afe_abc_mod2/AFE_control/afe_control/grid_voltage_phase_lock_loops/dq_pll/pll_stageB/double_integrator_observer/bounder2 ==
  data: u input; y output
function y = bounder(u)
    
    y = -pi + mod(u+3*pi,2*pi);
    
end

== matlab function grid_afe_n/afe_abc_mod2/AFE_control/afe_control/grid_voltage_sequences/grid_voltage_sampling_and_alpha_beta_transformation/v_abc2alphabeta ==
  data: v_abc input; alpha output; beta output
function [alpha,beta] = abc2alphabeta(v_abc)

alpha = 2/3*(v_abc(1) - 1/2*v_abc(2) - 1/2*v_abc(3));
beta  = 1/sqrt(3)*(v_abc(2) - v_abc(3));

end

== matlab function grid_afe_n/afe_abc_mod2/AFE_control/afe_control/grid_voltage_sequences/v_alphabeta2xieta/MATLAB Function ==
  data: alpha input; xi output; beta input; gamma input; eta output
function [xi,eta] = alphabeta2pos(alpha,beta,gamma)

    xi  =  alpha*cos(gamma) + beta*sin(gamma);
    eta = -alpha*sin(gamma) + beta*cos(gamma);

end

== matlab function grid_afe_n/afe_abc_mod1/AFE_control/afe_control/grid_voltage_phase_lock_loops/FHT-PLL/pll_stageB/bounder1 ==
  data: u input; y output
function y = bounder(u)
    y = -pi + mod(u+3*pi,2*pi);
end

== matlab function grid_afe_n/afe_abc_mod2/AFE_control/afe_control/grid_voltage_sequences/v_alphabeta2xieta/MATLAB Function1 ==
  data: alpha input; xi output; beta input; gamma input; eta output
function [xi,eta] = alphabeta2neg(alpha,beta,gamma)

    xi  = alpha*cos(gamma) - beta*sin(gamma);
    eta = alpha*sin(gamma) + beta*cos(gamma);

end

== matlab function grid_afe_n/afe_abc_mod2/AFE_control/afe_control/islanding_mode_detector/MATLAB Function ==
  data: alpha input; xi output; beta input; gamma input; eta output
function [xi,eta] = alphabeta2pos(alpha,beta,gamma)

    xi  =  alpha*cos(gamma) + beta*sin(gamma);
    eta = -alpha*sin(gamma) + beta*cos(gamma);

end
